simulink model "sf_aircraft_reu"  (R2025b)
settings: configuration reference "SharedConfig" (kept outside this file)
model workspace (MAT data in the model file):
  IsOuter = 0
  hydDEBOUNCE = 0
  hydMAXDELTA = 0
  hydMAXDIFF = 0
  hydMAXVAL = 0
  hydMINVAL = 0
  posDEBOUNCE = 0
  posMAXDELTA = 0
  posMAXDIFF = 0
  posMAXVAL = 0
  posMINVAL = 0
libraries: simulink x2, sf_aircraft_lib x2, slpidlib x1
settings Model: DataDictionary=sf_aircraft_dd.sldd  ParameterArgumentNames=IsOuter,hydDEBOUNCE,hydMAXDELTA,hydMAXDIFF,hydMAXVAL,hydMINVAL,posDEBOUNCE,posMAXDELTA,posMAXDIFF,posMAXVAL,posMINVAL  Creator=The MathWorks, Inc.  LastModifiedBy=The MathWorks, Inc.
settings ConfigSetRef: SourceName=SharedConfig

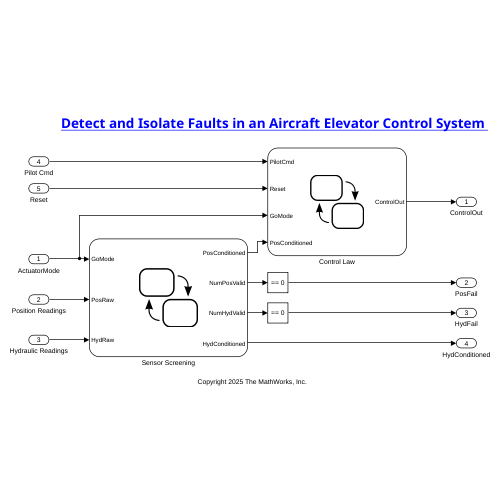
[thumbnail: Simulink's stored preview of the top-level diagram]
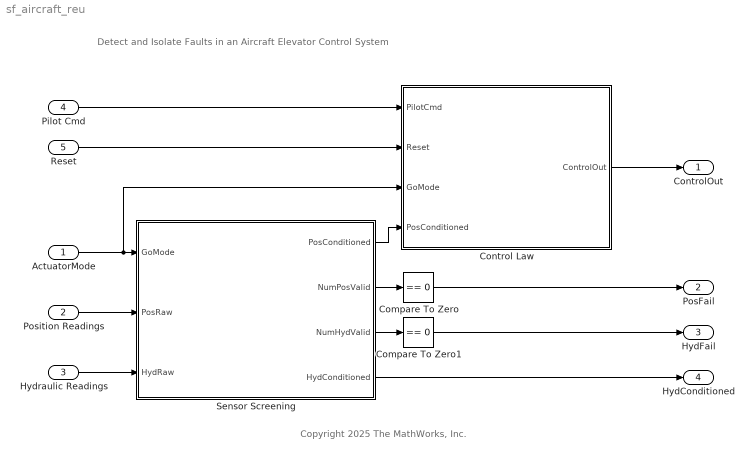
== system sf_aircraft_reu ==
  note: Copyright 2025 The MathWorks, Inc.
  note: Detect and Isolate Faults in an Aircraft Elevator Control System
  ActuatorMode : Inport
  Position Readings : Inport  Port=2
  Hydraulic Readings : Inport  Port=3
  Pilot Cmd : Inport  Port=4
  Reset : Inport  Port=5
  Compare To Zero : simulink/Logic and Bit Operations/Compare To Zero  relop===  OutDataTypeStr=boolean
  Compare To Zero1 : simulink/Logic and Bit Operations/Compare To Zero  relop===  OutDataTypeStr=boolean
  Control Law : Stateflow chart  TreatAsAtomicUnit=on  SystemSampleTime=.01
      settings: PortSchema="{\"entries\":[{\"content\":{\"sides\":[{\"content\":{\"connectorIds\":[\"In3\",\"In1\",\"In2\",\"In4\"]},\"type\":\"ConnectorPlacement.EquallySpacedRectSide\",\"uuid\":\"ece606a6-bc0a-4b92-b44f-2dcafb512ccb\"},{\"content\":{\"connectorIds\":[\"Out1\"],\"side\":\"RIGHT\"},\"type\":\"ConnectorPlacement.EquallySpacedRectSide\",\"uuid\":\"de4d026e-dcb3-40b5-9c55-5146ed3c61b6\"},{\"content\":{\"side\":\"TOP\"},\"type\":\"ConnectorPlacement.EquallySpacedRectSide\",\"uuid\":\"9f936c34-afb6-4efe-9ab7-85a351546cf6\"}]},\"type\":\"ConnectorPlacement.EquallySpacedConnector\",\"uuid\":\"52fde7bc-3686-4881-bcdd-530712a7f89a\"}],\"packageUris\":[\"http://schema.mathworks.com/mf0/Connector/R2020b\"],\"version\":\"1.0\"}"
  Sensor Screening : Stateflow chart  TreatAsAtomicUnit=on  SystemSampleTime=.01
      settings: PortSchema="{\"entries\":[{\"content\":{\"sides\":[{\"content\":{\"connectorIds\":[\"In1\",\"In2\",\"In3\"]},\"type\":\"ConnectorPlacement.EquallySpacedRectSide\",\"uuid\":\"5c402428-fbcf-4d9f-a371-2dc46bf4af26\"},{\"content\":{\"connectorIds\":[\"Out4\",\"Out1\",\"Out2\",\"Out3\"],\"side\":\"RIGHT\"},\"type\":\"ConnectorPlacement.EquallySpacedRectSide\",\"uuid\":\"112dc723-7752-4e13-a1ef-605e3503ae97\"},{\"content\":{\"side\":\"TOP\"},\"type\":\"ConnectorPlacement.EquallySpacedRectSide\",\"uuid\":\"ff1abd25-1ee5-41c2-adb1-2a88b98e965c\"}]},\"type\":\"ConnectorPlacement.EquallySpacedConnector\",\"uuid\":\"d1577901-0282-40d8-8f1a-34de190716bd\"}],\"packageUris\":[\"http://schema.mathworks.com/mf0/Connector/R2020b\"],\"version\":\"1.0\"}"
  ControlOut : Outport
  PosFail : Outport  Port=2
  HydFail : Outport  Port=3
  HydConditioned : Outport  Port=4
  wires:
  ActuatorMode/1 -> Control Law/2(GoMode), Sensor Screening/1(GoMode)
  Position Readings/1 -> Sensor Screening/2(PosRaw)
  Hydraulic Readings/1 -> Sensor Screening/3(HydRaw)
  Pilot Cmd/1 -> Control Law/3(PilotCmd)
  Sensor Screening/1(NumPosValid) -> Compare To Zero/1
  Sensor Screening/2(NumHydValid) -> Compare To Zero1/1
  Compare To Zero1/1 -> HydFail/1
  Compare To Zero/1 -> PosFail/1
  Sensor Screening/3(HydConditioned) -> HydConditioned/1
  Reset/1 -> Control Law/1(Reset)
  Control Law/1(ControlOut) -> ControlOut/1
  Sensor Screening/4(PosConditioned) -> Control Law/4(PosConditioned)

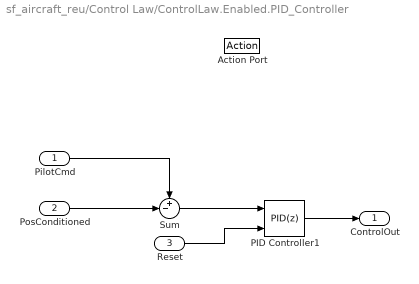
== system sf_aircraft_reu/Control Law/ControlLaw.Enabled.PID_Controller ==
  PilotCmd : Inport  OutDataTypeStr=double  PortDimensions=1
  PosConditioned : Inport  Port=2  OutDataTypeStr=double  PortDimensions=1
  Reset : Inport  Port=3  OutDataTypeStr=boolean  PortDimensions=1
  Action Port : ActionPort
      settings: CopyFcn=Stateflow.SLINSF.SimulinkMan.removeBlockPreDeleteFcn  PreDeleteFcn=Stateflow.SLINSF.SimulinkMan.unsafePredeleteFcn
  PID Controller1 : slpidlib/PID Controller  Controller=PID  Form=Parallel  TimeDomain=Discrete-time  UseExternalTs=off  SampleTime=-1  IntegratorMethod=Backward Euler  FilterMethod=Backward Euler  ControllerParametersSource=internal  P=0.0012  I=5.7e-4  UseKiTs=off  D=2.4e-4  UseExternalDerivativeSource=off  N=100  UseFilter=on  TunerSelectOption=Transfer Function Based (PID Tuner App)  InitialConditionSource=internal  InitialConditionForIntegrator=0  InitialConditionForFilter=0  DifferentiatorICPrevScaledInput=0  ExternalReset=rising  TrackingMode=off  Kt=1  LimitOutput=off  SatLimitsSource=internal  UpperSaturationLimit=inf  LowerSaturationLimit=-inf  LinearizeAsGain=on  AntiWindupMode=none  Kb=1  LimitIntegrator=off  UpperIntegratorSaturationLimit=inf  LowerIntegratorSaturationLimit=-inf  POutMin=[]  POutMax=[]  IOutMin=[]  IOutMax=[]  DOutMin=[]  DOutMax=[]  NOutMin=[]  NOutMax=[]  SumOutMin=[]  SumOutMax=[]  SaturationOutMin=[]  SaturationOutMax=[]  PParamMin=[]  PParamMax=[]  IParamMin=[]  IParamMax=[]  DParamMin=[]  DParamMax=[]  NParamMin=[]  NParamMax=[]  KbParamMin=[]  KbParamMax=[]  KtParamMin=[]  KtParamMax=[]  KbOutMin=[]  KbOutMax=[]  KtOutMin=[]  KtOutMax=[]  IntegratorOutMin=[]  IntegratorOutMax=[]  FilterOutMin=[]  FilterOutMax=[]  SumI1OutMin=[]  SumI1OutMax=[]  SumI2OutMin=[]  SumI2OutMax=[]  SumI3OutMin=[]  SumI3OutMax=[]  SumI4OutMin=[]  SumI4OutMax=[]  SumDOutMin=[]  SumDOutMax=[]  DifferentiatorOutMin=[]  DifferentiatorOutMax=[]  FilterDiffOutCoefMin=[]  FilterDiffOutCoefMax=[]  ReciprocalOutMin=[]  ReciprocalOutMax=[]  SumDenOutMin=[]  SumDenOutMax=[]  SumNumOutMin=[]  SumNumOutMax=[]  DivideOutMin=[]  DivideOutMax=[]  UdiffTsProdOutMin=[]  UdiffTsProdOutMax=[]  NTsProdOutMin=[]  NTsProdOutMax=[]  UintegralTsProdOutMin=[]  UintegralTsProdOutMax=[]  UngainTsProdOutMin=[]  UngainTsProdOutMax=[]  ClampingZeroOutDataTypeStr=Inherit: Inherit via back propagation  ClampingZeroOutMin=[]  ClampingZeroOutMax=[]  FilterDenConstantOutDataTypeStr=Inherit: Inherit via back propagation  FilterDenConstantOutMin=[]  FilterDenConstantOutMax=[]  PCopyOutDataTypeStr=Inherit: Inherit via back propagation  PCopyOutMin=[]  PCopyOutMax=[]  NCopyOutDataTypeStr=Inherit: Inherit via back propagation  NCopyOutMin=[]  NCopyOutMax=[]  IntegratorContinuousStateAttributes=''  IntegratorStateMustResolveToSignalObject=off  IntegratorRTWStateStorageClass=Auto  FilterContinuousStateAttributes=''  FilterStateMustResolveToSignalObject=off  FilterRTWStateStorageClass=Auto  ParallelPVariant=InternalParameters  IdealPVariant=Disabled  IVariant=InternalParameters  DVariant=InternalParameters  IntegratorVariant=Discrete  SatVariant=Disabled  AWVariant=Passthrough  PCopyVariant=Disabled  TRVariant=Disabled  FdbkBlocksVariant=Forward  IdealPFdbkVariant=Disabled  SatFdbkVariant=Disabled  DerivativeFilterVariant=BackwardEulerFilter  NVariant=InternalParameters  NCopyVariant=InternalParameters  FilterICVariant=InternalICsFilter  IntegratorICVariant=InternalICs  ExternalResetVariant=ExternalReset  TRSumVariant=Passthrough  SumFdbkVariant=Disabled  SumVariant=Sum_PID  TsampFilterVariant=InternalTs  TsampNgainVariant=Passthrough  TsampIntegralVariant=Disabled_SignalSpec  ExternalSaturationOutDataTypeStr=Inherit: Same as second input  DerivativeSourceVariant=ErrorSignal  PreIntVariant=InternalPreInt
  Sum : Sum  Inputs=+-|  SaturateOnIntegerOverflow=on
  ControlOut : Outport
  wires:
  PosConditioned/1 -> Sum/2
  PID Controller1/1 -> ControlOut/1
  Reset/1 -> PID Controller1/2
  PilotCmd/1 -> Sum/1
  Sum/1 -> PID Controller1/1

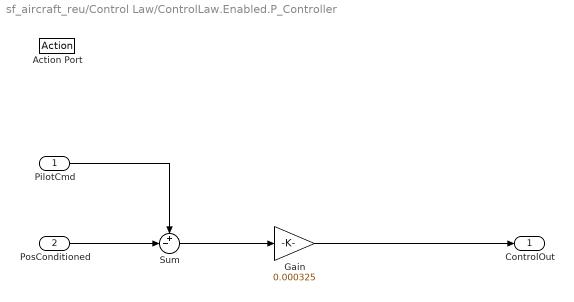
== system sf_aircraft_reu/Control Law/ControlLaw.Enabled.P_Controller ==
  PilotCmd : Inport
  PosConditioned : Inport  Port=2
  Action Port : ActionPort
      settings: CopyFcn=Stateflow.SLINSF.SimulinkMan.removeBlockPreDeleteFcn  PreDeleteFcn=Stateflow.SLINSF.SimulinkMan.unsafePredeleteFcn
  Gain : Gain  Gain=0.000325  SaturateOnIntegerOverflow=on  OutDataTypeStr=Inherit: Same as input  ParamDataTypeStr=Inherit: Same as input
  Sum : Sum  Inputs=+-|  SaturateOnIntegerOverflow=on
  ControlOut : Outport
  wires:
  Sum/1 -> Gain/1
  PosConditioned/1 -> Sum/2
  PilotCmd/1 -> Sum/1
  Gain/1 -> ControlOut/1

== stateflow chart sf_aircraft_reu/Sensor Screening ==
  settings: updateMethod=DISCRETE  sampleTime=.01
  state PositionSensorScreen [parallel]
    settings: executionOrder=1
  state HydraulicSensorScreen [parallel]
    settings: executionOrder=2
  data: GoMode input Enum: ActuatorModeType size=1; PosRaw input double size=3; HydRaw input double size=3; NumPosValid output uint8 size=1; NumHydValid output uint8 size=1; HydConditioned output double size=1; PosConditioned output double size=1

== stateflow chart sf_aircraft_reu/Control Law ==
  settings: updateMethod=DISCRETE  sampleTime=.01
  state ControlLaw
    state Enabled
      state PID_Controller
      state P_Controller
      (junction 68) -> PID_Controller [order 1] : [IsOuter]
      (default) -> (junction 68)
      (junction 68) -> P_Controller [order 2]
    state Disabled
      en,du:
      ControlOut = 0;
    (default) -> Disabled
    Disabled -> Enabled : [GoMode == ActuatorModeType.Active]
    Enabled -> Disabled : [GoMode ~= ActuatorModeType.Active]
  (default) -> ControlLaw
  data: sf_internal_action_state_placeholder_data local double size=1 =0; sf_internal_action_state_placeholder_data local double size=1 =0; Reset input boolean size=1; IsOuter parameter boolean; GoMode input Enum: ActuatorModeType size=1; ControlOut output; PilotCmd input double size=1; PosConditioned input double size=1
